simulink model "F104_lateral"  (R2026b)
settings: Solver=ode45  StopTime=20  MaxStep=0.01
undefined symbols (not defined in the file or in its folder): A, ail_amp, B, C, D, rud_amp, x0
settings Model: Creator=tensei  LastModifiedBy=tensei

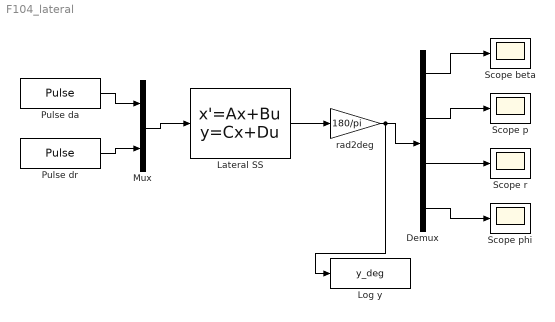
== system F104_lateral ==
  Demux : Demux
  Lateral SS : StateSpace  A=A  B=B  C=C  D=D  InitialCondition=x0
  Log y : ToWorkspace  VariableName=y_deg  SampleTime=-1
  Mux : Mux  Inputs=2
  Pulse da : DiscretePulseGenerator  PulseType=Time based  Amplitude=ail_amp  Period=20  PulseWidth=5
  Pulse dr : DiscretePulseGenerator  PulseType=Time based  Amplitude=rud_amp  Period=20  PulseWidth=5
  Scope beta : Scope
  Scope p : Scope
  Scope phi : Scope
  Scope r : Scope
  rad2deg : Gain  Gain=180/pi
  wires:
  Pulse da/1 -> Mux/1
  Pulse dr/1 -> Mux/2
  Mux/1 -> Lateral SS/1
  Lateral SS/1 -> rad2deg/1
  rad2deg/1 -> Demux/1, Log y/1
  Demux/1 -> Scope beta/1
  Demux/2 -> Scope p/1
  Demux/3 -> Scope r/1
  Demux/4 -> Scope phi/1
